simulink model "Lab5_p3_1_13b_Serial16"  (R2013b)
settings: Solver=FixedStepDiscrete  SolverMode=SingleTasking  StartTime=0.0  StopTime=inf  FixedStep=.05  RelTol=1e-3
libraries: simulink x3, arduinolib x1
settings Model: SimulationMode=external  ExtModeTrigDuration=2  Creator=Alec  LastModifiedBy=nding
settings OptimizationCC: ExpressionDepthLimit=2147483647  OptimizeModelRefInitCode=on  LifeSpan=1
settings DebuggingCC: SolverPrmCheckMsg=none  StateNameClashWarn=warning
settings HardwareCC: ProdBitPerInt=16  ProdBitPerPointer=8  ProdIntDivRoundTo=Zero  ProdEndianess=LittleEndian  ProdWordSize=8  ProdHWDeviceType=Atmel->AVR
settings RTWCC: SystemTargetFile=realtime.tlc  GenerateMakefile=off  TemplateMakefile=realtime.tmf  Description=Real-Time Toolbox  RTWVerbose=off  ProcessScript=realtime_make_rtw_hook
settings CodeAppCC: CustomSymbolStrType=$N$R$M  InternalIdentifier=Classic
settings STFCustomTargetCC: TargetLibSuffix=.a  GenerateSampleERTMain=on  ERTCustomFileBanners=on  SupportNonInlinedSFcns=off  SupportVariableSizeSignals=on  MATLABClassNameForMDSCustomization=Simulink.SoftwareTarget.ERTCustomization  GRTInterface=off  SystemTargetFile=realtime.tlc
settings ERTTargetCC: CodeReplacementLibrary=ANSI_C  GenerateSampleERTMain=on  ParMdlRefBuildCompliant=off  CompOptLevelCompliant=off  ConcurrentExecutionCompliant=off  CombineOutputUpdateFcns=off  ERTFirstTimeCompliant=off  SupportContinuousTime=on  SupportVariableSizeSignals=on  ModelStepFunctionPrototypeControlCompliant=off  CPPClassGenCompliant=off  ExtModeTransport=3  ExtModeMexFile=ext_serial_win32_comm  ExtModeMexArgs=0 21 115200  InlinedParameterPlacement=NonHierarchical  ERTSrcFileBannerTemplate=realtime_code_template.cgt  ERTHdrFileBannerTemplate=realtime_code_template.cgt  ERTDataSrcFileTemplate=realtime_code_template.cgt  ERTDataHdrFileTemplate=realtime_code_template.cgt  ERTCustomFileTemplate=realtime_file_process.tlc

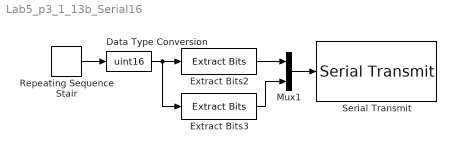
== system Lab5_p3_1_13b_Serial16 ==
  Data Type Conversion : DataTypeConversion  OutDataTypeStr=uint16
  Extract Bits2 : simulink/Logic and Bit Operations/Extract Bits  bitsToExtract=Upper half  numBits=8  bitIdxRange=[0 7]  outScalingMode=Treat bit field as an integer
  Extract Bits3 : simulink/Logic and Bit Operations/Extract Bits  bitsToExtract=Lower half  numBits=8  bitIdxRange=[0 7]  outScalingMode=Treat bit field as an integer
  Mux1 : Mux  Inputs=2
  Repeating Sequence Stair : simulink/Sources/Repeating Sequence Stair  OutValues=[-300:1:300]  tsamp=-1  OutMin=[]  OutMax=[]  OutDataTypeStr=double  OutputDataTypeScalingMode=double  OutDataType=fixdt(0,8)  ConRadixGroup=Best Precision: Vector-wise  OutScaling=2^-12
  Serial Transmit : arduinolib/Serial Transmit  portNumber=0
  wires:
  Repeating Sequence Stair/1 -> Data Type Conversion/1
  Extract Bits3/1 -> Mux1/2
  Mux1/1 -> Serial Transmit/1
  Data Type Conversion/1 -> Extract Bits3/1, Extract Bits2/1
  Extract Bits2/1 -> Mux1/1
